simulink model "PI_Controlled_Booster__YT_Ex_1"  (R2024a)
settings: Solver=VariableStepAuto  StartTime=0.0  StopTime=10  RelTol=1e-3
values from neighbouring files (symbols this model uses):
  C = 1000e-6    (= 0.001)    [New_RLC_finder_YT_Ex_1_for_physical_circuit.m]    (also in PI_Controlled_Booster_YT_EX_4.m = 0.00015; RLCFinder.m = 6.81055339577e-06; RLC_finder_YT_Ex_1.m = 0.00434027777778)
  L = 400e-6    (= 0.0004)    [New_RLC_finder_YT_Ex_1_for_physical_circuit.m]    (also in PI_Controlled_Booster_YT_EX_4.m = 0.045; RLCFinder.m = 0.0053344; RLC_finder_YT_Ex_1.m = 0.00144)
  R = Vref^2/Pload    (= 15)    [New_RLC_finder_YT_Ex_1_for_physical_circuit.m]    (also in PI_Controlled_Booster_YT_EX_4.m = 100; RLCFinder.m = 156.666666667; RLC_finder_YT_Ex_1.m = 1.152)
  Vin = 8.9    [New_RLC_finder_YT_Ex_1_for_physical_circuit.m]    (also in PI_Controlled_Booster_YT_EX_4.m = 15; RLCFinder.m = 8; RLC_finder_YT_Ex_1.m = 12)
  Vref = 15    [New_RLC_finder_YT_Ex_1_for_physical_circuit.m]    (also in RLC_finder_YT_Ex_1.m = 24)
libraries: spsSeriesRLCBranchLib x3, spsCurrentMeasurementLib x2, spsVoltageMeasurementLib x2, spsControlledVoltageSourceLib x1, spsDiodeLib x1, spsIGBTLib x1, slpidlib x1, spsPWMGeneratorDCDCLib x1, sps_lib x1
settings Model: Creator=Razowan  LastModifiedBy=Razowan
settings DataIOCC: ReturnWorkspaceOutputs=off

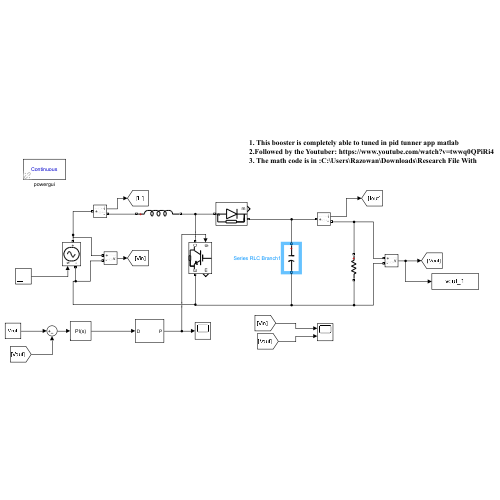
[thumbnail: Simulink's stored preview of the top-level diagram]
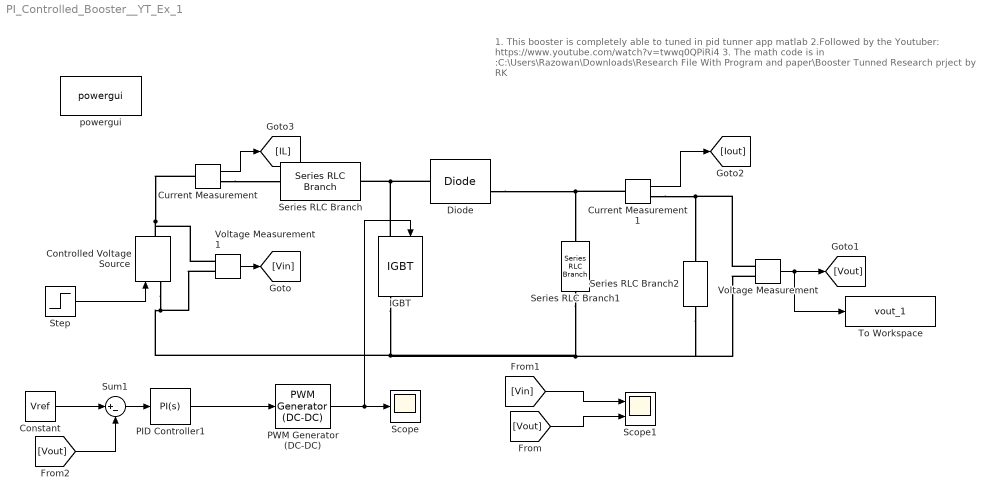
== system PI_Controlled_Booster__YT_Ex_1 ==
  note: 1. This booster is completely able to tuned in pid tunner app matlab
      | 2.Followed by the Youtuber: https://www.youtube.com/watch?v=twwq0QPiRi4
      | 3. The math code is in :C:\Users\Razowan\Downloads\Research File With Program and paper\Booster Tunned Research prject by RK
  Constant : Constant  Value=Vref
  Controlled Voltage Source : spsControlledVoltageSourceLib/Controlled Voltage Source  Initialize=on  Source_Type=AC  Amplitude=0  Phase=0  Frequency=0  Measurements=None
  Current Measurement : spsCurrentMeasurementLib/Current Measurement  PhasorSimulation=off  OutputType=Complex  PSBequivalent=0
  Current Measurement1 : spsCurrentMeasurementLib/Current Measurement  PhasorSimulation=off  OutputType=Complex  PSBequivalent=0
  Diode : spsDiodeLib/Diode  Ron=0.001  Lon=0  Vf=0.8  IC=0  UseSnubber=0  Rs=500  Cs=250e-9  Measurements=on
  IGBT : spsIGBTLib/IGBT  Ron=0.001  Lon=0  Vf=1  Tf=1e-6  Tt=2e-6  IC=0  Rs=1e5  Cs=inf  Measurements=on
  PID Controller1 : slpidlib/PID Controller  Controller=PI  Form=Parallel  TimeDomain=Continuous-time  UseExternalTs=off  SampleTime=-1  IntegratorMethod=Forward Euler  FilterMethod=Forward Euler  ControllerParametersSource=internal  P=1  I=1  UseKiTs=off  D=0  UseExternalDerivativeSource=off  N=100  UseFilter=on  TunerSelectOption=Transfer Function Based (PID Tuner App)  InitialConditionSource=internal  InitialConditionForIntegrator=0  InitialConditionForFilter=0  DifferentiatorICPrevScaledInput=0  ExternalReset=none  TrackingMode=off  Kt=1  LimitOutput=off  SatLimitsSource=internal  UpperSaturationLimit=inf  LowerSaturationLimit=-inf  LinearizeAsGain=on  AntiWindupMode=none  Kb=1  LimitIntegrator=off  UpperIntegratorSaturationLimit=inf  LowerIntegratorSaturationLimit=-inf  POutMin=[]  POutMax=[]  IOutMin=[]  IOutMax=[]  DOutMin=[]  DOutMax=[]  NOutMin=[]  NOutMax=[]  SumOutMin=[]  SumOutMax=[]  SaturationOutMin=[]  SaturationOutMax=[]  PParamMin=[]  PParamMax=[]  IParamMin=[]  IParamMax=[]  DParamMin=[]  DParamMax=[]  NParamMin=[]  NParamMax=[]  KbParamMin=[]  KbParamMax=[]  KtParamMin=[]  KtParamMax=[]  KbOutMin=[]  KbOutMax=[]  KtOutMin=[]  KtOutMax=[]  IntegratorOutMin=[]  IntegratorOutMax=[]  FilterOutMin=[]  FilterOutMax=[]  SumI1OutMin=[]  SumI1OutMax=[]  SumI2OutMin=[]  SumI2OutMax=[]  SumI3OutMin=[]  SumI3OutMax=[]  SumI4OutMin=[]  SumI4OutMax=[]  SumDOutMin=[]  SumDOutMax=[]  DifferentiatorOutMin=[]  DifferentiatorOutMax=[]  FilterDiffOutCoefMin=[]  FilterDiffOutCoefMax=[]  ReciprocalOutMin=[]  ReciprocalOutMax=[]  SumDenOutMin=[]  SumDenOutMax=[]  SumNumOutMin=[]  SumNumOutMax=[]  DivideOutMin=[]  DivideOutMax=[]  UdiffTsProdOutMin=[]  UdiffTsProdOutMax=[]  NTsProdOutMin=[]  NTsProdOutMax=[]  UintegralTsProdOutMin=[]  UintegralTsProdOutMax=[]  UngainTsProdOutMin=[]  UngainTsProdOutMax=[]  ClampingZeroOutDataTypeStr=Inherit: Inherit via back propagation  ClampingZeroOutMin=[]  ClampingZeroOutMax=[]  FilterDenConstantOutDataTypeStr=Inherit: Inherit via back propagation  FilterDenConstantOutMin=[]  FilterDenConstantOutMax=[]  PCopyOutDataTypeStr=Inherit: Inherit via back propagation  PCopyOutMin=[]  PCopyOutMax=[]  NCopyOutDataTypeStr=Inherit: Inherit via back propagation  NCopyOutMin=[]  NCopyOutMax=[]  IntegratorContinuousStateAttributes=''  IntegratorStateMustResolveToSignalObject=off  IntegratorRTWStateStorageClass=Auto  FilterContinuousStateAttributes=''  FilterStateMustResolveToSignalObject=off  FilterRTWStateStorageClass=Auto  ParallelPVariant=InternalParameters  IdealPVariant=Disabled  IVariant=InternalParameters  DVariant=Disabled  IntegratorVariant=Continuous  SatVariant=Disabled  AWVariant=Passthrough  PCopyVariant=Disabled  TRVariant=Disabled  FdbkBlocksVariant=Forward  IdealPFdbkVariant=Disabled  SatFdbkVariant=Disabled  DerivativeFilterVariant=Disabled  NVariant=Disabled  NCopyVariant=Disabled_SignalSpec  FilterICVariant=Disabled  IntegratorICVariant=InternalICs  ExternalResetVariant=Disabled  TRSumVariant=Passthrough  SumFdbkVariant=Disabled  SumVariant=Sum_PI  TsampFilterVariant=InternalTs  TsampNgainVariant=Passthrough  TsampIntegralVariant=Disabled_SignalSpec  ExternalSaturationOutDataTypeStr=Inherit: Same as second input  DerivativeSourceVariant=Disabled
  PWM Generator (DC-DC) : spsPWMGeneratorDCDCLib/PWM Generator (DC-DC)  Fsw=fs  Ts=0
  Scope : Scope
  Scope1 : Scope  NumInputPorts=2
  Series RLC Branch : spsSeriesRLCBranchLib/Series RLC Branch  LConnTagsString=__new0  RConnTagsString=__new0  BranchType=L  Resistance=1  Inductance=L  SetiL0=off  InitialCurrent=0  Capacitance=1e-6  Setx0=off  InitialVoltage=0  Measurements=None
  Series RLC Branch1 : spsSeriesRLCBranchLib/Series RLC Branch  LConnTagsString=__new0  RConnTagsString=__new0  BranchType=C  Resistance=1  Inductance=L  SetiL0=off  InitialCurrent=0  Capacitance=C  Setx0=off  InitialVoltage=0  Measurements=None
  Series RLC Branch2 : spsSeriesRLCBranchLib/Series RLC Branch  LConnTagsString=__new0  RConnTagsString=__new0  BranchType=R  Resistance=R  Inductance=L  SetiL0=off  InitialCurrent=0  Capacitance=1e-6  Setx0=off  InitialVoltage=0  Measurements=None
  Step : Step  Before=Vin  After=12  SampleTime=0
  Sum1 : Sum  Inputs=|+-
  To Workspace : ToWorkspace  VariableName=vout_1  SaveFormat=Timeseries  SampleTime=-1
  Voltage Measurement : spsVoltageMeasurementLib/Voltage Measurement  PhasorSimulation=off  OutputType=Complex  PSBequivalent=0
  Voltage Measurement1 : spsVoltageMeasurementLib/Voltage Measurement  PhasorSimulation=off  OutputType=Complex  PSBequivalent=0
  powergui : sps_lib/powergui  Priority=1  SimulationMode=Continuous  SampleTime=1e-6  frequency=60  Iterations=50  frequencyindice=0  Pbase=100e6  ErrMax=1e-4  UnitsV=kV  UnitsW=MW  buscounter=0  FunctionMessages=off  echomessages=off  EnableUseOfTLC=off  CurrentSourceSwitches=off  DisableSnubberDevices=off  DisableRonSwitches=off  DisableVfSwitches=off  DisplayEquations=off  AutomaticDiscreteSolvers=off  SolverType=Tustin/Backward Euler (TBE)  Interpol=off  ExternalGateDelay=off  methode=off  Ts=100  x0status=blocks  SPID=on  SwTol=0  HookPort=off  NonlinearTolerance=1e-4  nMaxIteration=100  ContinueOnMaxIteration=off  RestoreLinks=warning  ResistiveCurrentMeasurement=off  Frange=[0:2:500]  Ylog=off  Xlog=on  ShowGrid=off  save=off  variable=ZData  structure=0  ZoomFFT=off  StartTime=0.0  cycles=1  DisplayStyle=1  fundamental=60  FreqAxis=off  MaxFrequency=1000  frequencyindicesteady=1  RmsSteady=1  display=off
  wires:
  Voltage Measurement1/1 -> [Vin]
  Current Measurement/1 -> [IL]
  Current Measurement1/1 -> [Iout]
  PWM Generator (DC-DC)/1 -> Scope/1, IGBT/1
  [Vout] -> Scope1/2
  [Vin] -> Scope1/1
  Sum1/1 -> PID Controller1/1
  Constant/1 -> Sum1/1
  [Vout] -> Sum1/2
  Step/1 -> Controlled Voltage Source/1
  Voltage Measurement/1 -> To Workspace/1, [Vout]
  PID Controller1/1 -> PWM Generator (DC-DC)/1
  connections:
  Current Measurement/RConn1 -- Series RLC Branch/LConn1
  Current Measurement/LConn1 -- Voltage Measurement1/LConn1 -- Controlled Voltage Source/RConn1
  Diode/LConn1 -- IGBT/LConn1 -- Series RLC Branch/RConn1
  IGBT/RConn1 -- Voltage Measurement/LConn2 -- Series RLC Branch2/RConn1 -- Series RLC Branch1/RConn1 -- Controlled Voltage Source/LConn1 -- Voltage Measurement1/LConn2
  Diode/RConn1 -- Current Measurement1/LConn1 -- Series RLC Branch1/LConn1
  Voltage Measurement/LConn1 -- Current Measurement1/RConn1 -- Series RLC Branch2/LConn1
